simulink model "single_phase_dab"  (R2026b)
settings: Solver=ode23tb  StopTime=param.sim.simlength  FixedStep=param.glb_time.tc  MaxStep=param.glb_time.tc
values from neighbouring files (symbols this model uses):
  param = struct()    [init_model.m]
libraries: fl_lib x22, nesl_utility x15, discrete_time_low_pass_filter x7, lithium_ion_battery x2, pi_ctrl x2, full_bridge_ideal_switch x2, full_bridge_mosfet_based_with_thermal_model x2, full_bridge_mosfet_based_with_thermal_model_zvs x2, dab_single_phase_pwm_modulator x1, single_phase_transformer x1
(part 2 of 2)

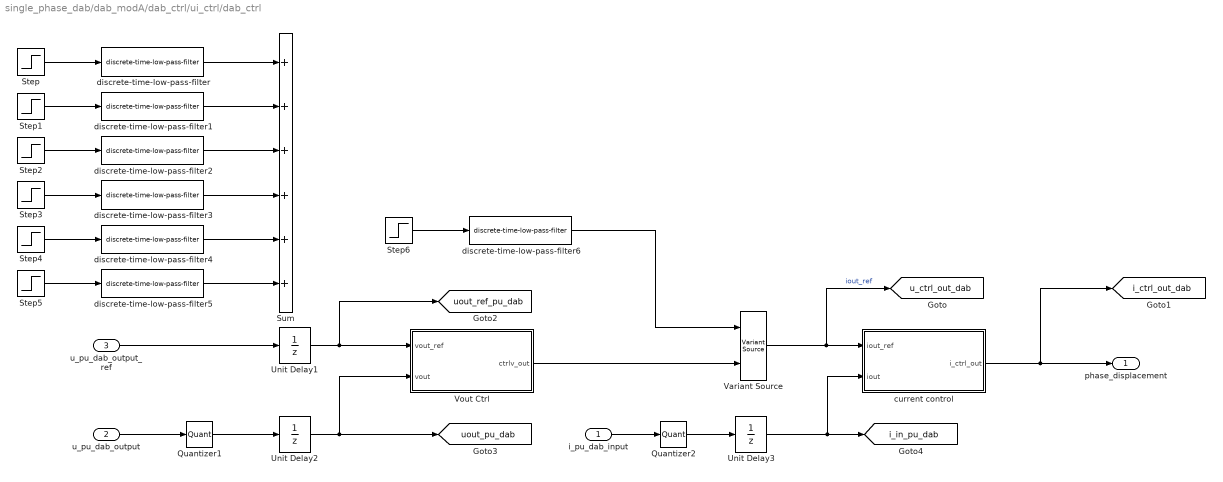
== system single_phase_dab/dab_modA/dab_ctrl/ui_ctrl/dab_ctrl ==
  i_pu_dab_input : Inport
  u_pu_dab_output : Inport  Port=2
  u_pu_dab_output_ref : Inport  Port=3
  Quantizer1 : Quantizer  QuantizationInterval=param.meas.adc12_quantization
  Quantizer2 : Quantizer  QuantizationInterval=param.meas.adc12_quantization
  Step : Step  Time=0.05  FinalValue=0.25
  Step1 : Step  Time=0.4  FinalValue=0.75
  Step2 : Step  Time=0.6  FinalValue=0.25
  Step3 : Step  Time=0.8  FinalValue=-1
  Step4 : Step  FinalValue=-0.75
  Step5 : Step  Time=1.25  FinalValue=-0.5
  Step6 : Step  Time=param.dab.bench.t_step  InitialValue=param.dab.bench.i_ref0  FinalValue=param.dab.bench.i_ref1
  Sum : Sum  Inputs=++++++
  Unit Delay1 : UnitDelay  SampleTime=-1
  Unit Delay2 : UnitDelay  SampleTime=-1
  Unit Delay3 : UnitDelay  SampleTime=-1
  Variant Source : VariantSource  VariantControls={true, false}
  Vout Ctrl : Subsystem
  current control : Subsystem
  discrete-time-low-pass-filter{,1..5} (6 alike) : discrete_time_low_pass_filter/discrete-time-low-pass-filter  tau=0.02  ts=param.glb_time.ts_dab
  discrete-time-low-pass-filter6 : discrete_time_low_pass_filter/discrete-time-low-pass-filter  tau=param.dab.bench.tau_ref  ts=param.glb_time.ts_dab
  phase_displacement : Outport
  tag scope: i_ctrl_out_dab=global, i_in_pu_dab=global, u_ctrl_out_dab=global, uout_pu_dab=global, uout_ref_pu_dab=global
  wires:
  Vout Ctrl/1(ctrlv_out) -> Variant Source/2
  Variant Source/1 -> [u_ctrl_out_dab], current control/1(iout_ref)  "iout_ref"
  i_pu_dab_input/1 -> Quantizer2/1
  current control/1(i_ctrl_out) -> phase_displacement/1, [i_ctrl_out_dab]
  Unit Delay3/1 -> current control/2(iout), [i_in_pu_dab]
  Unit Delay2/1 -> [uout_pu_dab], Vout Ctrl/2(vout)
  Unit Delay1/1 -> Vout Ctrl/1(vout_ref), [uout_ref_pu_dab]
  u_pu_dab_output/1 -> Quantizer1/1
  Step/1 -> discrete-time-low-pass-filter/1
  Step1/1 -> discrete-time-low-pass-filter1/1
  Step2/1 -> discrete-time-low-pass-filter2/1
  Step3/1 -> discrete-time-low-pass-filter3/1
  Step4/1 -> discrete-time-low-pass-filter4/1
  Step5/1 -> discrete-time-low-pass-filter5/1
  discrete-time-low-pass-filter/1 -> Sum/1
  discrete-time-low-pass-filter1/1 -> Sum/2
  discrete-time-low-pass-filter2/1 -> Sum/3
  discrete-time-low-pass-filter3/1 -> Sum/4
  discrete-time-low-pass-filter4/1 -> Sum/5
  discrete-time-low-pass-filter5/1 -> Sum/6
  u_pu_dab_output_ref/1 -> Unit Delay1/1
  Quantizer1/1 -> Unit Delay2/1
  Quantizer2/1 -> Unit Delay3/1
  Step6/1 -> discrete-time-low-pass-filter6/1
  discrete-time-low-pass-filter6/1 -> Variant Source/1

== system single_phase_dab/dab_modA/dab_ctrl/ui_ctrl/scopes ==
  Bus Creator : BusCreator  Inputs=2
  Bus Creator1 : BusCreator  Inputs=2
  dab-tracking : Scope  NumInputPorts=2
      settings: ActiveDisplayYMinimum=-0.7264395439314022  ActiveDisplayYMaximum=2.2614067014075516  DataLoggingVariableName=ScopeData7
  u_ctrl_out_dab/i_ctrl_out_dab : Scope  NumInputPorts=2
      settings: ActiveDisplayYMinimum=-1.2812486231311795  ActiveDisplayYMaximum=1.531237608180616
  wires:
  Bus Creator1/1 -> dab-tracking/2
  Bus Creator/1 -> dab-tracking/1
  [i_ctrl_out_dab] -> u_ctrl_out_dab/i_ctrl_out_dab/2  "i_ctrl_out_dab"
  [i_in_pu_dab] -> Bus Creator1/2  "i_in_pu_dab"
  [uout_ref_pu_dab] -> Bus Creator/1  "uout_ref_pu_dab"
  [u_ctrl_out_dab] -> u_ctrl_out_dab/i_ctrl_out_dab/1  "u_ctrl_out_dab"
  [u_ctrl_out_dab] -> Bus Creator1/1  "u_ctrl_out_dab"
  [uout_pu_dab] -> Bus Creator/2  "uout_pu_dab"

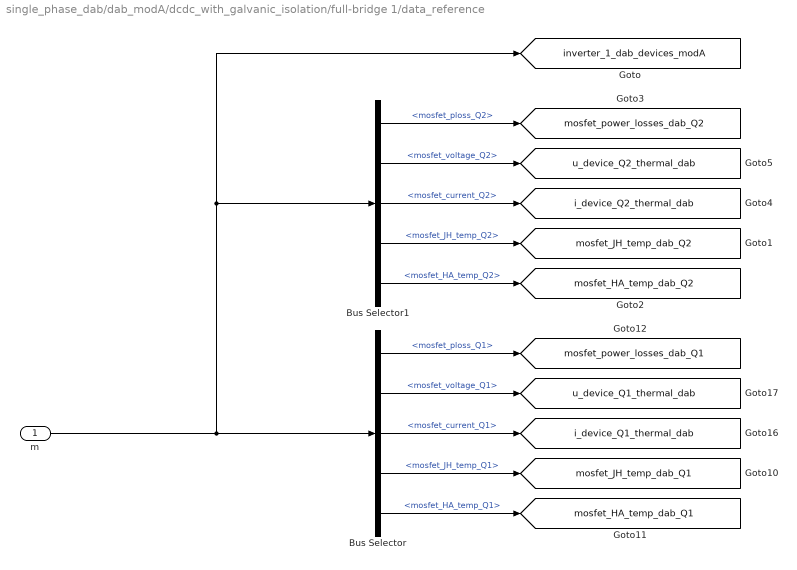
== system single_phase_dab/dab_modA/dcdc_with_galvanic_isolation/full-bridge 1/data_reference ==
  m : Inport
  Bus Selector : BusSelector  OutputSignals=mosfet_ploss_Q1,mosfet_voltage_Q1,mosfet_current_Q1,mosfet_JH_temp_Q1,mosfet_HA_temp_Q1
  Bus Selector1 : BusSelector  OutputSignals=mosfet_ploss_Q2,mosfet_voltage_Q2,mosfet_current_Q2,mosfet_JH_temp_Q2,mosfet_HA_temp_Q2
  tag scope: i_device_Q1_thermal_dab=global, i_device_Q2_thermal_dab=global, inverter_1_dab_devices_modA=global, mosfet_HA_temp_dab_Q1=global, mosfet_HA_temp_dab_Q2=global, mosfet_JH_temp_dab_Q1=global, mosfet_JH_temp_dab_Q2=global, mosfet_power_losses_dab_Q1=global, mosfet_power_losses_dab_Q2=global, u_device_Q1_thermal_dab=global, u_device_Q2_thermal_dab=global
  wires:
  Bus Selector/1 -> [mosfet_power_losses_dab_Q1]  "<mosfet_ploss_Q1>"
  Bus Selector1/3 -> [i_device_Q2_thermal_dab]  "<mosfet_current_Q2>"
  Bus Selector1/2 -> [u_device_Q2_thermal_dab]  "<mosfet_voltage_Q2>"
  Bus Selector1/5 -> [mosfet_HA_temp_dab_Q2]  "<mosfet_HA_temp_Q2>"
  Bus Selector/4 -> [mosfet_JH_temp_dab_Q1]  "<mosfet_JH_temp_Q1>"
  Bus Selector/5 -> [mosfet_HA_temp_dab_Q1]  "<mosfet_HA_temp_Q1>"
  Bus Selector1/4 -> [mosfet_JH_temp_dab_Q2]  "<mosfet_JH_temp_Q2>"
  Bus Selector/3 -> [i_device_Q1_thermal_dab]  "<mosfet_current_Q1>"
  Bus Selector/2 -> [u_device_Q1_thermal_dab]  "<mosfet_voltage_Q1>"
  Bus Selector1/1 -> [mosfet_power_losses_dab_Q2]  "<mosfet_ploss_Q2>"
  m/1 -> Bus Selector/1, Bus Selector1/1, [inverter_1_dab_devices_modA]

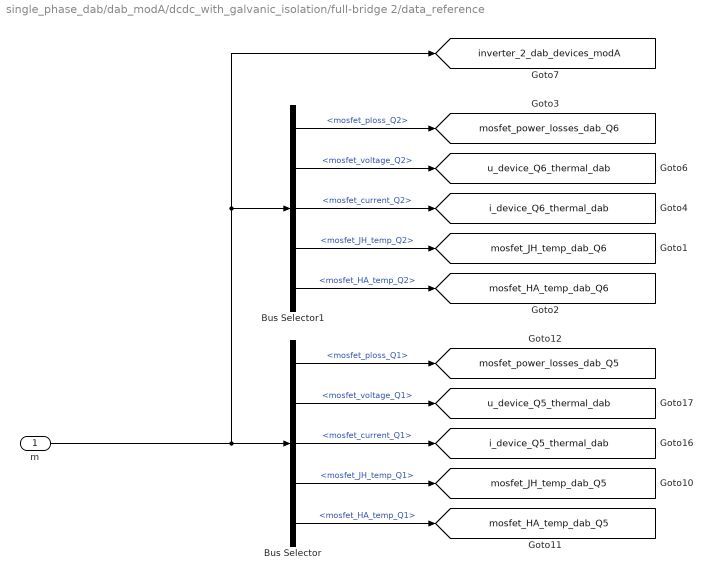
== system single_phase_dab/dab_modA/dcdc_with_galvanic_isolation/full-bridge 2/data_reference ==
  m : Inport
  Bus Selector : BusSelector  OutputSignals=mosfet_ploss_Q1,mosfet_voltage_Q1,mosfet_current_Q1,mosfet_JH_temp_Q1,mosfet_HA_temp_Q1
  Bus Selector1 : BusSelector  OutputSignals=mosfet_ploss_Q2,mosfet_voltage_Q2,mosfet_current_Q2,mosfet_JH_temp_Q2,mosfet_HA_temp_Q2
  tag scope: i_device_Q5_thermal_dab=global, i_device_Q6_thermal_dab=global, inverter_2_dab_devices_modA=global, mosfet_HA_temp_dab_Q5=global, mosfet_HA_temp_dab_Q6=global, mosfet_JH_temp_dab_Q5=global, mosfet_JH_temp_dab_Q6=global, mosfet_power_losses_dab_Q5=global, mosfet_power_losses_dab_Q6=global, u_device_Q5_thermal_dab=global, u_device_Q6_thermal_dab=global
  wires:
  Bus Selector1/3 -> [i_device_Q6_thermal_dab]  "<mosfet_current_Q2>"
  Bus Selector1/4 -> [mosfet_JH_temp_dab_Q6]  "<mosfet_JH_temp_Q2>"
  Bus Selector/3 -> [i_device_Q5_thermal_dab]  "<mosfet_current_Q1>"
  Bus Selector1/1 -> [mosfet_power_losses_dab_Q6]  "<mosfet_ploss_Q2>"
  m/1 -> [inverter_2_dab_devices_modA], Bus Selector1/1, Bus Selector/1
  Bus Selector/4 -> [mosfet_JH_temp_dab_Q5]  "<mosfet_JH_temp_Q1>"
  Bus Selector1/2 -> [u_device_Q6_thermal_dab]  "<mosfet_voltage_Q2>"
  Bus Selector/1 -> [mosfet_power_losses_dab_Q5]  "<mosfet_ploss_Q1>"
  Bus Selector/5 -> [mosfet_HA_temp_dab_Q5]  "<mosfet_HA_temp_Q1>"
  Bus Selector/2 -> [u_device_Q5_thermal_dab]  "<mosfet_voltage_Q1>"
  Bus Selector1/5 -> [mosfet_HA_temp_dab_Q6]  "<mosfet_HA_temp_Q2>"

== system single_phase_dab/dab_modA/dab_ctrl/ui_ctrl/dab_ctrl/Vout Ctrl ==
  vout_ref : Inport
  vout : Inport  Port=2
  pi_ctrl : pi_ctrl/pi_ctrl  kp=param.dab.ctrl.kp_udc  ki=param.dab.ctrl.ki_udc  ts=param.glb_time.ts_dab  lim_up=2  lim_down=-2
  ctrlv_out : Outport
  wires:
  vout_ref/1 -> pi_ctrl/1
  vout/1 -> pi_ctrl/2
  pi_ctrl/1 -> ctrlv_out/1

== system single_phase_dab/dab_modA/dab_ctrl/ui_ctrl/dab_ctrl/current control ==
  iout_ref : Inport
  iout : Inport  Port=2
  Gain : Gain  Gain=param.dab.mod.k_ff
  i_out_dab_tracking : Scope  NumInputPorts=3
      settings: ActiveDisplayYMinimum=-1.1754092261904745  ActiveDisplayYMaximum=1.8310081845238102  DataLoggingVariableName=ScopeData12
  pi_ctrl : pi_ctrl/pi_ctrl  kp=param.dab.ctrl.kp_idc  ki=param.dab.ctrl.ki_idc  ts=param.glb_time.ts_dab  lim_up=1  lim_down=-1
  i_ctrl_out : Outport
  wires:
  iout_ref/1 -> pi_ctrl/1, i_out_dab_tracking/1, Gain/1  "i_out_dab_ref"
  iout/1 -> pi_ctrl/2, i_out_dab_tracking/2  "i_out_dab"
  pi_ctrl/1 -> i_ctrl_out/1, i_out_dab_tracking/3  "i_ctrl_out"
  Gain/1 -> pi_ctrl/3
